simulink subsystem "PowerSystemRefAeronomie"  (R2024b)
settings: Solver=VariableStepAuto  StartTime=0.0  StopTime=10.0  RelTol=1e-3
undefined symbols (not defined in the file or in its folder): ess, mot, powerplant, propel, pxf_diagram_options, SimIn, tc
libraries: simulink x2, slpidlib x1, matrix_library x1
(part 1 of 3)
settings Model: Creator=drhill  LastModifiedBy=edison
settings SolverCC: AlgebraicLoopSolver=TrustRegion
settings OptimizationCC: ReuseModelBlockBuffer=off
settings DebuggingCC: UnconnectedInputMsg=warning  UnconnectedOutputMsg=warning  UnconnectedLineMsg=warning
settings ModelReferenceCC: EnableRefExpFcnMdlSchedulingChecks=on
settings RTWCC: GPUComputeCapability=3.5  DLArmComputeVersion=19.05

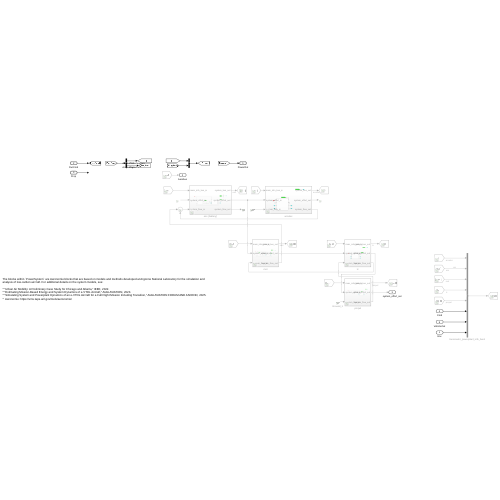
[thumbnail: Simulink's stored preview of the top-level diagram]
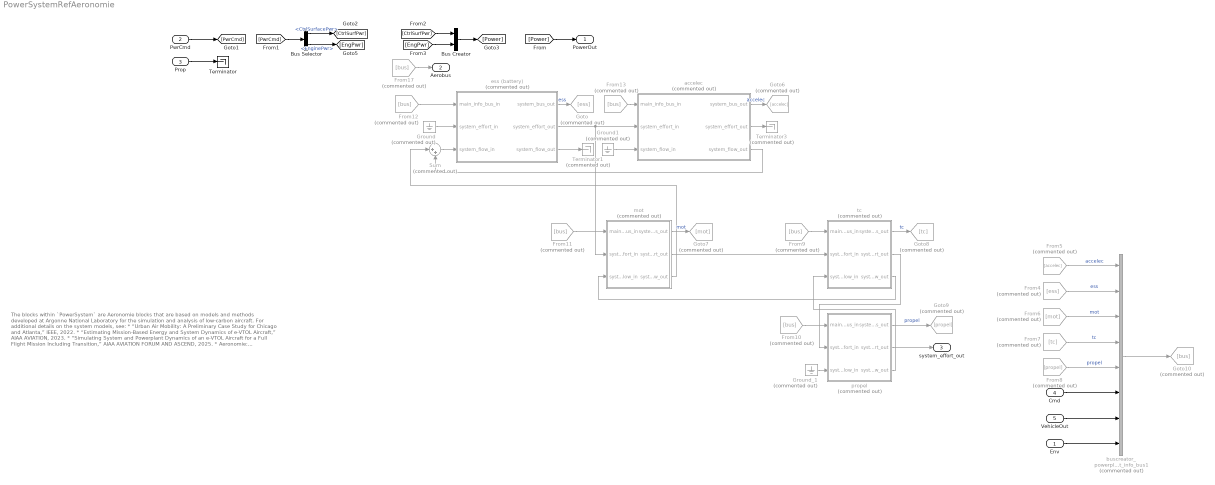
== system PowerSystemRefAeronomie ==
  note: The blocks within `PowerSystem` are Aeronomie blocks that are based on models and methods developed at Argonne National Laboratory for the simulation and analysis of low-carbon aircraft. For additional details on the system models, see:
      |
      | * “Urban Air Mobility: A Preliminary Case Study for Chicago and Atlanta,” IEEE, 2022.
      | * “Estimating Mission-Based Energy and System Dynamics of e-VTOL Aircraft,” AIAA AVIATION, 2023.
      | * “Simulating System and Powerplant Dynamics of an e-VTOL Aircraft for a Full Flight Mission Including Transition,” AIAA AVIATION FORUM AND ASCEND, 2025.
      | * Aeronomie: https://vms.taps.anl.gov/tools/aeronomie/
  Env : Inport
  PwrCmd : Inport  Port=2  OutDataTypeStr=Bus: BUS_POWER_SYSTEM_IN
  Prop : Inport  Port=3  OutDataTypeStr=Bus: BUS_PROP_ACTUATOR
  Cmd : Inport  Port=4
  VehicleOut : Inport  Port=5
  Bus Creator : BusCreator  Inputs=2  OutDataTypeStr=Bus: BUS_POWER_SYSTEM_OUT
  Bus Selector : BusSelector  OutputSignals=CtrlSurfacePwr,EnginePwr
  From{9..13,17} (6 alike) : From  Commented=on  GotoTag=bus
  From4 : From  Commented=on  GotoTag=ess
  From5 : From  Commented=on  GotoTag=accelec
  From6 : From  Commented=on  GotoTag=mot
  From7 : From  Commented=on  GotoTag=tc
  From8 : From  Commented=on  GotoTag=propel
  Goto : Goto  Commented=on  GotoTag=ess
  Goto10 : Goto  Commented=on  GotoTag=bus
  Goto6 : Goto  Commented=on  GotoTag=accelec
  Goto7 : Goto  Commented=on  GotoTag=mot
  Goto8 : Goto  Commented=on  GotoTag=tc
  Goto9 : Goto  Commented=on  GotoTag=propel
  Ground : Ground  Commented=on
  Ground1 : Ground  Commented=on
  Ground_1 : Ground  Commented=on
  Sum : Sum  Commented=on  Inputs=|++
  Terminator : Terminator
  Terminator1 : Terminator  Commented=on
  Terminator3 : Terminator  Commented=on
  accelec : Subsystem  Commented=on
  buscreator_powerplant_info_bus1 : BusCreator  Commented=on  Inputs=8
  ess (battery) : Subsystem  Commented=on
  mot : Subsystem  Commented=on
  propel : Subsystem  Commented=on
  tc : Subsystem  Commented=on
  PowerOut : Outport  OutDataTypeStr=Bus: BUS_POWER_SYSTEM_OUT  VectorParamsAs1DForOutWhenUnconnected=off
  Aerobus : Outport  Port=2
  system_effort_out : Outport  Port=3
  wires:
  mot/2(system_effort_out) -> tc/2(system_effort_in)
  Ground_1/1 -> propel/3(system_flow_in)
  tc/3(system_flow_out) -> mot/3(system_flow_in)
  tc/2(system_effort_out) -> propel/2(system_effort_in)
  propel/3(system_flow_out) -> tc/3(system_flow_in)
  Bus Creator/1 -> [Power]
  [Power] -> PowerOut/1
  PwrCmd/1 -> [PwrCmd]
  [PwrCmd] -> Bus Selector/1
  Bus Selector/1 -> [CtrlSurfPwr]  "<CtrlSurfacePwr>"
  [CtrlSurfPwr] -> Bus Creator/1
  [EngPwr] -> Bus Creator/2
  Ground/1 -> ess (battery)/2(system_effort_in)
  Prop/1 -> Terminator/1
  ess (battery)/3(system_flow_out) -> Terminator1/1
  Bus Selector/2 -> [EngPwr]  "<EnginePwr>"
  ess (battery)/2(system_effort_out) -> mot/2(system_effort_in), accelec/2(system_effort_in)
  Ground1/1 -> accelec/3(system_flow_in)
  Sum/1 -> ess (battery)/3(system_flow_in)
  accelec/3(system_flow_out) -> Sum/2
  accelec/2(system_effort_out) -> Terminator3/1
  accelec/1(system_bus_out) -> Goto6/1  "accelec"
  From5/1 -> buscreator_powerplant_info_bus1/1  "accelec"
  From4/1 -> buscreator_powerplant_info_bus1/2  "ess"
  From6/1 -> buscreator_powerplant_info_bus1/3  "mot"
  mot/1(system_bus_out) -> Goto7/1  "mot"
  tc/1(system_bus_out) -> Goto8/1  "tc"
  propel/1(system_bus_out) -> Goto9/1  "propel"
  From7/1 -> buscreator_powerplant_info_bus1/4  "tc"
  From8/1 -> buscreator_powerplant_info_bus1/5  "propel"
  From9/1 -> tc/1(main_info_bus_in)
  From10/1 -> propel/1(main_info_bus_in)
  From11/1 -> mot/1(main_info_bus_in)
  Cmd/1 -> buscreator_powerplant_info_bus1/6
  Env/1 -> buscreator_powerplant_info_bus1/8
  From12/1 -> ess (battery)/1(main_info_bus_in)
  From13/1 -> accelec/1(main_info_bus_in)
  ess (battery)/1(system_bus_out) -> Goto/1  "ess"
  propel/2(system_effort_out) -> system_effort_out/1
  From17/1 -> Aerobus/1
  VehicleOut/1 -> buscreator_powerplant_info_bus1/7
  buscreator_powerplant_info_bus1/1 -> Goto10/1
  mot/3(system_flow_out) -> Sum/1

== system PowerSystemRefAeronomie/accelec ==
  main_info_bus_in : Inport
  system_effort_in : Inport  Port=2
  system_flow_in : Inport  Port=3
  Ground_1 : Ground
  Terminator_1 : Terminator
  plant : Subsystem
      mask Display: disp('accelec_plant_const_pwrloss_volt_in_nokey.slx')
  system_bus_out : Outport
  system_effort_out : Outport  Port=2
  system_flow_out : Outport  Port=3
  wires:
  main_info_bus_in/1 -> plant/1(aInport--1)
  plant/1(outport-system_info_bus) -> [plant]
  plant/3(out-effort-6) -> system_effort_out/1
  plant/4(out-flow-7) -> system_flow_out/1
  system_effort_in/1 -> plant/3(in-effort-2)
  system_flow_in/1 -> plant/4(in-flow-3)
  [plant] -> system_bus_out/1  "plant"
  Ground_1/1 -> plant/2(aInport--2)
  plant/2(aOutport--2) -> Terminator_1/1

== system PowerSystemRefAeronomie/ess (battery) ==
  main_info_bus_in : Inport
  system_effort_in : Inport  Port=2
  system_flow_in : Inport  Port=3
  buscreator_system_bus_out1 : BusCreator  Inputs=2
  ctrl : Subsystem
      mask Display: disp('ess_ctrl_pngv_map_anl_PI_cstr.slx')
  memoryctrl : Memory
  plant : Subsystem
      mask Display: disp('ess_plant_pngv_map_anl_PI_cstr.slx')
  system_bus_out : Outport
  system_effort_out : Outport  Port=2
  system_flow_out : Outport  Port=3
  wires:
  ctrl/1(outport-system_info_bus) -> [ctrl]  "system_info_bus"
  ctrl/2(outport-ctrl_bus) -> memoryctrl/1  "ctrl_bus"
  main_info_bus_in/1 -> ctrl/1(inport-main_info_bus-1), plant/1(aInport--1)  "main_info_bus"
  plant/2(outport-plant_bus) -> ctrl/2(aInport--2)  "plant_bus"
  memoryctrl/1 -> plant/2(aInport--2)  "ctrl_bus"
  plant/1(outport-system_info_bus) -> [plant]  "system_info_bus"
  plant/3(out-effort-12) -> system_effort_out/1  "effort"
  plant/4(out-flow-13) -> system_flow_out/1  "flow"
  system_effort_in/1 -> plant/3(in-effort-1)  "effort"
  system_flow_in/1 -> plant/4(in-flow-2)  "flow"
  buscreator_system_bus_out1/1 -> system_bus_out/1  "system_info_bus"
  [ctrl] -> buscreator_system_bus_out1/1  "ctrl"
  [plant] -> buscreator_system_bus_out1/2  "plant"

== system PowerSystemRefAeronomie/mot ==
  main_info_bus_in : Inport
  system_effort_in : Inport  Port=2
  system_flow_in : Inport  Port=3
  buscreator_system_bus_out1 : BusCreator  Inputs=2
  ctrl : Subsystem
  memoryctrl : Memory
  plant : Subsystem
      mask Display: disp('mot_plant_map_Pelec_funTW_volt_in.slx')
  system_bus_out : Outport
  system_effort_out : Outport  Port=2
  system_flow_out : Outport  Port=3
  wires:
  ctrl/1(system_bus_out) -> [ctrl]  "system_info_bus"
  ctrl/2(local_info_bus_out) -> memoryctrl/1  "ctrl_bus"
  main_info_bus_in/1 -> ctrl/1(main_info_bus_in), plant/1(aInport--1)  "main_info_bus"
  plant/2(outport-plant_bus) -> ctrl/2(local_info_bus_in)  "plant_bus"
  memoryctrl/1 -> plant/2(inport-ctrl_bus-2)  "ctrl_bus"
  plant/1(outport-system_info_bus) -> [plant]  "system_info_bus"
  plant/3(out-effort-7) -> system_effort_out/1  "effort"
  plant/4(out-flow-8) -> system_flow_out/1  "flow"
  system_effort_in/1 -> plant/3(in-effort-2)  "effort"
  system_flow_in/1 -> plant/4(in-flow-3)  "flow"
  buscreator_system_bus_out1/1 -> system_bus_out/1  "system_info_bus"
  [ctrl] -> buscreator_system_bus_out1/1  "ctrl"
  [plant] -> buscreator_system_bus_out1/2  "plant"

== system PowerSystemRefAeronomie/propel ==
  main_info_bus_in : Inport
  system_effort_in : Inport  Port=2
  system_flow_in : Inport  Port=3
  Ground_1 : Ground
  Terminator_1 : Terminator
  plant : Subsystem
      mask Display: disp('propel_plant_uas.slx')
  system_bus_out : Outport
  system_effort_out : Outport  Port=2
  system_flow_out : Outport  Port=3
  wires:
  main_info_bus_in/1 -> plant/1(inport-main_info_bus-1)
  plant/1(outport-system_info_bus) -> [plant]
  plant/3(out-effort-5) -> system_effort_out/1
  plant/4(out-flow-6) -> system_flow_out/1
  system_effort_in/1 -> plant/3(in-effort-4)
  system_flow_in/1 -> plant/4(in-flow-5)
  [plant] -> system_bus_out/1  "plant"
  Ground_1/1 -> plant/2(aInport--2)
  plant/2(aOutport--2) -> Terminator_1/1

== system PowerSystemRefAeronomie/tc ==
  main_info_bus_in : Inport
  system_effort_in : Inport  Port=2
  system_flow_in : Inport  Port=3
  Ground_1 : Ground
  Terminator_1 : Terminator
  plant : Subsystem
      mask Display: disp('tc_plant_map_trqloss_funTW.slx')
  system_bus_out : Outport
  system_effort_out : Outport  Port=2
  system_flow_out : Outport  Port=3
  wires:
  main_info_bus_in/1 -> plant/1(aInport--1)
  plant/1(outport-system_info_bus) -> [plant]
  plant/3(out-effort-7) -> system_effort_out/1
  plant/4(out-flow-8) -> system_flow_out/1
  system_effort_in/1 -> plant/3(in-effort-1)
  system_flow_in/1 -> plant/4(in-flow-2)
  [plant] -> system_bus_out/1  "plant"
  Ground_1/1 -> plant/2(aInport--2)
  plant/2(aOutport--2) -> Terminator_1/1

== system PowerSystemRefAeronomie/accelec/plant ==
  aInport--1 : Inport
  aInport--2 : Inport  Port=2
  in-effort-2 : Inport  Port=3
  in-flow-3 : Inport  Port=4
  Ground_1 : Ground
  Ground_2 : Ground
  Terminator_1 : Terminator
  Terminator_2 : Terminator
  accelec_plant_const_pwrloss_volt_in_nokey : Subsystem
  parameter_out : Subsystem
  parameter_selection : Subsystem
  outport-system_info_bus : Outport
  aOutport--2 : Outport  Port=2
  out-effort-6 : Outport  Port=3
  out-flow-7 : Outport  Port=4
  wires:
  parameter_out/1(outport-system_info_bus) -> outport-system_info_bus/1
  accelec_plant_const_pwrloss_volt_in_nokey/1(accelec_plant_volt_in_simu) -> parameter_out/1(inport-accelec_plant_volt_in_simu)
  accelec_plant_const_pwrloss_volt_in_nokey/2(accelec_plant_pwr_simu) -> parameter_out/2(inport-accelec_plant_pwr_simu)
  accelec_plant_const_pwrloss_volt_in_nokey/3(accelec_plant_curr_in_simu) -> parameter_out/3(inport-accelec_plant_curr_in_simu)
  accelec_plant_const_pwrloss_volt_in_nokey/4(accelec_plant_volt_out_simu) -> parameter_out/4(inport-accelec_plant_volt_out_simu)
  accelec_plant_const_pwrloss_volt_in_nokey/5(accelec_plant_curr_out_simu) -> parameter_out/5(inport-accelec_plant_curr_out_simu)
  in-effort-2/1 -> accelec_plant_const_pwrloss_volt_in_nokey/2(accelec_volt_in)
  in-flow-3/1 -> accelec_plant_const_pwrloss_volt_in_nokey/3(accelec_curr_out)
  accelec_plant_const_pwrloss_volt_in_nokey/6(accelec_volt_out) -> out-effort-6/1
  accelec_plant_const_pwrloss_volt_in_nokey/7(accelec_curr_in) -> out-flow-7/1
  aInport--1/1 -> Terminator_1/1
  aInport--2/1 -> Terminator_2/1
  Ground_1/1 -> accelec_plant_const_pwrloss_volt_in_nokey/1(drv_key_on_dmd_simu)
  Ground_2/1 -> aOutport--2/1

== system PowerSystemRefAeronomie/ess (battery)/ctrl ==
  inport-main_info_bus-1 : Inport
  aInport--2 : Inport  Port=2
  Terminator_1 : Terminator
  ess_ctrl_pngv_map_anl_PI_cstr : Subsystem
  parameter_out : Subsystem
  parameter_selection : Subsystem
  outport-system_info_bus : Outport
  outport-ctrl_bus : Outport  Port=2
  wires:
  inport-main_info_bus-1/1 -> parameter_selection/1(inport-main_info_bus-1)
  parameter_out/1(outport-system_info_bus) -> outport-system_info_bus/1
  parameter_out/2(outport-ctrl_bus) -> outport-ctrl_bus/1
  ess_ctrl_pngv_map_anl_PI_cstr/1(ess_ctrl_pwr_max_pro_simu) -> parameter_out/1(inport-ess_ctrl_pwr_max_pro_simu)
  ess_ctrl_pngv_map_anl_PI_cstr/2(ess_ctrl_pwr_max_reg_simu) -> parameter_out/2(inport-ess_ctrl_pwr_max_reg_simu)
  ess_ctrl_pngv_map_anl_PI_cstr/3(ess_ctrl_curr_max_pro_simu) -> parameter_out/3(inport-ess_ctrl_curr_max_pro_simu)
  ess_ctrl_pngv_map_anl_PI_cstr/4(ess_ctrl_curr_max_reg_simu) -> parameter_out/4(inport-ess_ctrl_curr_max_reg_simu)
  parameter_selection/1(outport-ess_plant_volt_out_simu-1) -> ess_ctrl_pngv_map_anl_PI_cstr/1(ess_volt_out)
  parameter_selection/2(outport-ess_plant_curr_out_simu-2) -> ess_ctrl_pngv_map_anl_PI_cstr/2(ess_curr_out)
  parameter_selection/3(outport-ess_plant_soc_simu-3) -> ess_ctrl_pngv_map_anl_PI_cstr/3(ess_soc)
  aInport--2/1 -> Terminator_1/1

== system PowerSystemRefAeronomie/ess (battery)/plant ==
  aInport--1 : Inport
  aInport--2 : Inport  Port=2
  in-effort-1 : Inport  Port=3
  in-flow-2 : Inport  Port=4
  Terminator_1 : Terminator
  Terminator_2 : Terminator
  ess_plant_pngv_map_anl_PI_cstr : Subsystem
  parameter_out : Subsystem
  parameter_selection : Subsystem
  outport-system_info_bus : Outport
  outport-plant_bus : Outport  Port=2
  out-effort-12 : Outport  Port=3
  out-flow-13 : Outport  Port=4
  wires:
  parameter_out/1(outport-system_info_bus) -> outport-system_info_bus/1
  parameter_out/2(outport-plant_bus) -> outport-plant_bus/1
  ess_plant_pngv_map_anl_PI_cstr/1(ess_plant_soc_simu) -> parameter_out/1(inport-ess_plant_soc_simu)
  ess_plant_pngv_map_anl_PI_cstr/10(ess_plant_heat_out_simu) -> parameter_out/10(inport-ess_plant_heat_out_simu)
  ess_plant_pngv_map_anl_PI_cstr/11(ess_plant_impedance_simu) -> parameter_out/11(inport-ess_plant_impedance_simu)
  ess_plant_pngv_map_anl_PI_cstr/2(ess_plant_curr_out_simu) -> parameter_out/2(inport-ess_plant_curr_out_simu)
  ess_plant_pngv_map_anl_PI_cstr/3(ess_plant_volt_out_simu) -> parameter_out/3(inport-ess_plant_volt_out_simu)
  ess_plant_pngv_map_anl_PI_cstr/4(ess_plant_voc_simu) -> parameter_out/4(inport-ess_plant_voc_simu)
  ess_plant_pngv_map_anl_PI_cstr/5(ess_plant_rint_simu) -> parameter_out/5(inport-ess_plant_rint_simu)
  ess_plant_pngv_map_anl_PI_cstr/6(ess_plant_rpol1_simu) -> parameter_out/6(inport-ess_plant_rpol1_simu)
  ess_plant_pngv_map_anl_PI_cstr/7(ess_plant_rpol2_simu) -> parameter_out/7(inport-ess_plant_rpol2_simu)
  ess_plant_pngv_map_anl_PI_cstr/8(ess_plant_curr_pol1_simu) -> parameter_out/8(inport-ess_plant_curr_pol1_simu)
  ess_plant_pngv_map_anl_PI_cstr/9(ess_plant_curr_pol2_simu) -> parameter_out/9(inport-ess_plant_curr_pol2_simu)
  in-effort-1/1 -> ess_plant_pngv_map_anl_PI_cstr/1(ess_volt_in)
  in-flow-2/1 -> ess_plant_pngv_map_anl_PI_cstr/2(ess_curr_out)
  ess_plant_pngv_map_anl_PI_cstr/12(ess_volt_out) -> out-effort-12/1
  ess_plant_pngv_map_anl_PI_cstr/13(ess_curr_in) -> out-flow-13/1
  aInport--1/1 -> Terminator_1/1
  aInport--2/1 -> Terminator_2/1

== system PowerSystemRefAeronomie/mot/ctrl ==
  main_info_bus_in : Inport
  local_info_bus_in : Inport  Port=2
  buscreator_system_bus_out1 : BusCreator  Inputs=3
  cmd : Subsystem
      mask Display: disp('mot_ctrl_cmd_map_Pelec_funTW_volt_in.slx')
  cstr : Subsystem
      mask Display: disp('mot_ctrl_cstr_map_Pelec_funTW_volt_in.slx')
  dmd : Subsystem
      mask Display: disp('mot_ctrl_dmd_uas.slx')
  system_bus_out : Outport
  local_info_bus_out : Outport  Port=2
  wires:
  dmd/1(outport-system_info_bus) -> [dmd]
  dmd/2(outport-dmd_bus) -> cmd/4(aInport--4), cstr/3(aInport--3)
  [local_info_bus] -> dmd/2(aInport--2)
  [main_info_bus] -> dmd/1(inport-main_info_bus-1)
  cstr/1(outport-system_info_bus) -> [cstr]
  cstr/2(outport-cstr_bus) -> cmd/3(aInport--3)
  [local_info_bus] -> cstr/2(aInport--2)
  [main_info_bus] -> cstr/1(inport-main_info_bus-1)
  cmd/1(outport-system_info_bus) -> local_info_bus_out/1, [cmd]
  [local_info_bus] -> cmd/2(aInport--2)
  [main_info_bus] -> cmd/1(inport-main_info_bus-1)
  main_info_bus_in/1 -> [main_info_bus]
  local_info_bus_in/1 -> [local_info_bus]
  buscreator_system_bus_out1/1 -> system_bus_out/1
  [cmd] -> buscreator_system_bus_out1/1  "cmd"
  [cstr] -> buscreator_system_bus_out1/2  "cstr"
  [dmd] -> buscreator_system_bus_out1/3  "dmd"

== system PowerSystemRefAeronomie/mot/plant ==
  aInport--1 : Inport
  inport-ctrl_bus-2 : Inport  Port=2
  in-effort-2 : Inport  Port=3
  in-flow-3 : Inport  Port=4
  Ground_1 : Ground
  Terminator_1 : Terminator
  mot_plant_map_Pelec_funTW_volt_in : Subsystem
  parameter_out : Subsystem
  parameter_selection : Subsystem
  outport-system_info_bus : Outport
  outport-plant_bus : Outport  Port=2
  out-effort-7 : Outport  Port=3
  out-flow-8 : Outport  Port=4
  wires:
  inport-ctrl_bus-2/1 -> parameter_selection/2(inport-ctrl_bus-2)
  parameter_out/1(outport-system_info_bus) -> outport-system_info_bus/1
  parameter_out/2(outport-plant_bus) -> outport-plant_bus/1
  mot_plant_map_Pelec_funTW_volt_in/1(mot_plant_spd_out_simu) -> parameter_out/1(inport-mot_plant_spd_out_simu)
  mot_plant_map_Pelec_funTW_volt_in/2(mot_plant_curr_in_simu) -> parameter_out/2(inport-mot_plant_curr_in_simu)
  mot_plant_map_Pelec_funTW_volt_in/3(mot_plant_volt_in_simu) -> parameter_out/3(inport-mot_plant_volt_in_simu)
  mot_plant_map_Pelec_funTW_volt_in/4(mot_plant_cmd_simu) -> parameter_out/4(inport-mot_plant_cmd_simu)
  mot_plant_map_Pelec_funTW_volt_in/5(mot_plant_trq_out_simu) -> parameter_out/5(inport-mot_plant_trq_out_simu)
  mot_plant_map_Pelec_funTW_volt_in/6(mot_plant_temp_coeff_simu) -> parameter_out/6(inport-mot_plant_temp_coeff_simu)
  parameter_selection/1(outport-mot_ctrl_cmd_simu-1) -> mot_plant_map_Pelec_funTW_volt_in/1(mot_ctrl_cmd_simu)
  in-effort-2/1 -> mot_plant_map_Pelec_funTW_volt_in/2(voltage)
  in-flow-3/1 -> mot_plant_map_Pelec_funTW_volt_in/3(spd)
  mot_plant_map_Pelec_funTW_volt_in/7(mot_trq_out mot_inertia_out) -> out-effort-7/1
  mot_plant_map_Pelec_funTW_volt_in/8(mot_current_out) -> out-flow-8/1
  aInport--1/1 -> Terminator_1/1
  Ground_1/1 -> parameter_selection/1(Inport_1)

== system PowerSystemRefAeronomie/propel/plant ==
  inport-main_info_bus-1 : Inport
  aInport--2 : Inport  Port=2
  in-effort-4 : Inport  Port=3
  in-flow-5 : Inport  Port=4
  Ground_1 : Ground
  Terminator_1 : Terminator
  parameter_out : Subsystem
  parameter_selection : Subsystem
  propel_plant_uas : Subsystem
  outport-system_info_bus : Outport
  aOutport--2 : Outport  Port=2
  out-effort-5 : Outport  Port=3
  out-flow-6 : Outport  Port=4
  wires:
  propel_plant_uas/7(propel_plant_effort_dn) -> parameter_out/6(propel_plant_effort_dn1)
  parameter_selection/4(tc_plant_trq_out_simu) -> propel_plant_uas/4(tc_plant_trq_out_simu)
  parameter_selection/5(AdvanceRatio) -> propel_plant_uas/6(AdvanceRatio)
  inport-main_info_bus-1/1 -> parameter_selection/1(inport-main_info_bus-1)
  parameter_out/1(outport-system_info_bus) -> outport-system_info_bus/1
  propel_plant_uas/1(propel_plant_speed_simu) -> parameter_out/1(inport-propel_plant_speed_simu)
  propel_plant_uas/2(propel_plant_pwr_in_simu) -> parameter_out/2(inport-propel_plant_pwr_in_simu)
  propel_plant_uas/3(propel_plant_pwr_out_simu) -> parameter_out/3(inport-propel_plant_pwr_out_simu)
  propel_plant_uas/4(propel_plant_thrust_simu) -> parameter_out/4(inport-propel_plant_thrust_simu)
  parameter_selection/1(outport-env_plant_density_simu-1) -> propel_plant_uas/1(env_plant_density_simu)
  parameter_selection/2(outport-tc_plant_inertia_out_simu-2) -> propel_plant_uas/2(tc_plant_inertia_out_simu)
  parameter_selection/3(outport-eqnmotion_plant_linvel_simu-3) -> propel_plant_uas/3(eqnmotion_plant_linvel_simu)
  in-flow-5/1 -> propel_plant_uas/5(flow-in)
  propel_plant_uas/5(propel_plant_effort) -> out-effort-5/1, parameter_out/5(propel_plant_effort)
  propel_plant_uas/6(propel_plant_speed_out_simu) -> out-flow-6/1
  aInport--2/1 -> Terminator_1/1
  Ground_1/1 -> aOutport--2/1

== system PowerSystemRefAeronomie/tc/plant ==
  aInport--1 : Inport
  aInport--2 : Inport  Port=2
  in-effort-1 : Inport  Port=3
  in-flow-2 : Inport  Port=4
  Ground_1 : Ground
  Terminator_1 : Terminator
  Terminator_2 : Terminator
  parameter_out : Subsystem
  parameter_selection : Subsystem
  tc_plant_map_trqloss_funTW : Subsystem
  outport-system_info_bus : Outport
  aOutport--2 : Outport  Port=2
  out-effort-7 : Outport  Port=3
  out-flow-8 : Outport  Port=4
  wires:
  parameter_out/1(outport-system_info_bus) -> outport-system_info_bus/1
  tc_plant_map_trqloss_funTW/1(tc_plant_trq_in_simu) -> parameter_out/1(inport-tc_plant_trq_in_simu)
  tc_plant_map_trqloss_funTW/2(tc_plant_trq_out_simu) -> parameter_out/2(inport-tc_plant_trq_out_simu)
  tc_plant_map_trqloss_funTW/3(tc_plant_spd_in_simu) -> parameter_out/3(inport-tc_plant_spd_in_simu)
  tc_plant_map_trqloss_funTW/4(tc_plant_spd_out_simu) -> parameter_out/4(inport-tc_plant_spd_out_simu)
  tc_plant_map_trqloss_funTW/5(tc_plant_inertia_in_simu) -> parameter_out/5(inport-tc_plant_inertia_in_simu)
  tc_plant_map_trqloss_funTW/6(tc_plant_inertia_out_simu) -> parameter_out/6(inport-tc_plant_inertia_out_simu)
  in-effort-1/1 -> tc_plant_map_trqloss_funTW/1(tc_trq_in tc_inertia_in)
  in-flow-2/1 -> tc_plant_map_trqloss_funTW/2(tc_spd_out)
  tc_plant_map_trqloss_funTW/7(tc_trq_out) -> out-effort-7/1
  tc_plant_map_trqloss_funTW/8(tc_spd_in) -> out-flow-8/1
  aInport--2/1 -> Terminator_2/1
  Ground_1/1 -> aOutport--2/1
  aInport--1/1 -> Terminator_1/1

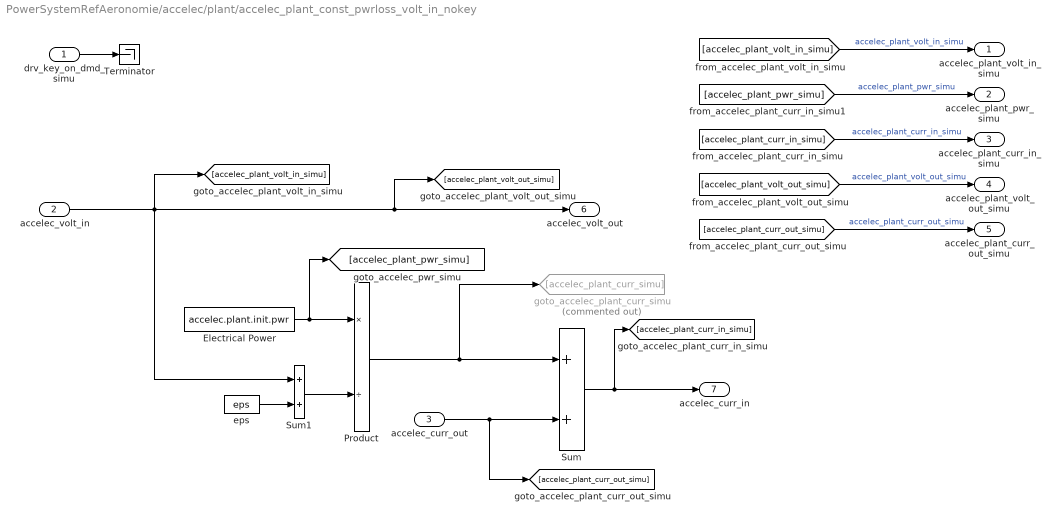
== system PowerSystemRefAeronomie/accelec/plant/accelec_plant_const_pwrloss_volt_in_nokey ==
  drv_key_on_dmd_simu : Inport
  accelec_volt_in : Inport  Port=2
  accelec_curr_out : Inport  Port=3
  Electrical Power : Constant  Value=accelec.plant.init.pwr
  Product : Product  Inputs=*/  InputSameDT=on  SaturateOnIntegerOverflow=on  OutDataTypeStr=Inherit: Same as first input
  Sum : Sum  InputSameDT=on  SaturateOnIntegerOverflow=on  OutDataTypeStr=Inherit: Same as first input
  Sum1 : Sum  InputSameDT=on  SaturateOnIntegerOverflow=on  OutDataTypeStr=Inherit: Same as first input
  Terminator : Terminator
  eps : Constant  Value=eps
  goto_accelec_plant_curr_simu : Goto  Commented=on  GotoTag=accelec_plant_curr_simu
  accelec_plant_volt_in_simu : Outport  VectorParamsAs1DForOutWhenUnconnected=off
  accelec_plant_pwr_simu : Outport  Port=2  VectorParamsAs1DForOutWhenUnconnected=off
  accelec_plant_curr_in_simu : Outport  Port=3  VectorParamsAs1DForOutWhenUnconnected=off
  accelec_plant_volt_out_simu : Outport  Port=4  VectorParamsAs1DForOutWhenUnconnected=off
  accelec_plant_curr_out_simu : Outport  Port=5  VectorParamsAs1DForOutWhenUnconnected=off
  accelec_volt_out : Outport  Port=6  VectorParamsAs1DForOutWhenUnconnected=off
  accelec_curr_in : Outport  Port=7  VectorParamsAs1DForOutWhenUnconnected=off
  wires:
  drv_key_on_dmd_simu/1 -> Terminator/1
  Electrical Power/1 -> Product/1, [accelec_plant_pwr_simu]
  [accelec_plant_volt_out_simu] -> accelec_plant_volt_out_simu/1  "accelec_plant_volt_out_simu"
  [accelec_plant_curr_out_simu] -> accelec_plant_curr_out_simu/1  "accelec_plant_curr_out_simu"
  [accelec_plant_curr_in_simu] -> accelec_plant_curr_in_simu/1  "accelec_plant_curr_in_simu"
  Sum1/1 -> Product/2
  Sum/1 -> accelec_curr_in/1, [accelec_plant_curr_in_simu]
  accelec_curr_out/1 -> Sum/2, [accelec_plant_curr_out_simu]
  Product/1 -> Sum/1, goto_accelec_plant_curr_simu/1
  eps/1 -> Sum1/2
  [accelec_plant_volt_in_simu] -> accelec_plant_volt_in_simu/1  "accelec_plant_volt_in_simu"
  accelec_volt_in/1 -> accelec_volt_out/1, [accelec_plant_volt_out_simu], [accelec_plant_volt_in_simu], Sum1/1
  [accelec_plant_pwr_simu] -> accelec_plant_pwr_simu/1  "accelec_plant_pwr_simu"

== system PowerSystemRefAeronomie/accelec/plant/parameter_out ==
  inport-accelec_plant_volt_in_simu : Inport
  inport-accelec_plant_pwr_simu : Inport  Port=2
  inport-accelec_plant_curr_in_simu : Inport  Port=3
  inport-accelec_plant_volt_out_simu : Inport  Port=4
  inport-accelec_plant_curr_out_simu : Inport  Port=5
  Ground_1 : Ground
  Toworkspace-accelec_plant_curr_in_simu : ToWorkspace  VariableName=accelec_plant_curr_in_simu  SampleTime=pxf_diagram_options.workspace_sample_time
      settings: Decimation=pxf_diagram_options.decimation
  Toworkspace-accelec_plant_curr_out_simu : ToWorkspace  VariableName=accelec_plant_curr_out_simu  SampleTime=pxf_diagram_options.workspace_sample_time
      settings: Decimation=pxf_diagram_options.decimation
  Toworkspace-accelec_plant_pwr_simu : ToWorkspace  VariableName=accelec_plant_pwr_simu  SampleTime=pxf_diagram_options.workspace_sample_time
      settings: Decimation=pxf_diagram_options.decimation
  Toworkspace-accelec_plant_volt_in_simu : ToWorkspace  VariableName=accelec_plant_volt_in_simu  SampleTime=pxf_diagram_options.workspace_sample_time
      settings: Decimation=pxf_diagram_options.decimation
  Toworkspace-accelec_plant_volt_out_simu : ToWorkspace  VariableName=accelec_plant_volt_out_simu  SampleTime=pxf_diagram_options.workspace_sample_time
      settings: Decimation=pxf_diagram_options.decimation
  outport-system_info_bus : Outport
  wires:
  inport-accelec_plant_volt_in_simu/1 -> Toworkspace-accelec_plant_volt_in_simu/1
  inport-accelec_plant_pwr_simu/1 -> Toworkspace-accelec_plant_pwr_simu/1
  inport-accelec_plant_curr_in_simu/1 -> Toworkspace-accelec_plant_curr_in_simu/1
  inport-accelec_plant_volt_out_simu/1 -> Toworkspace-accelec_plant_volt_out_simu/1
  inport-accelec_plant_curr_out_simu/1 -> Toworkspace-accelec_plant_curr_out_simu/1
  Ground_1/1 -> outport-system_info_bus/1

== system PowerSystemRefAeronomie/accelec/plant/parameter_selection ==

== system PowerSystemRefAeronomie/ess (battery)/ctrl/ess_ctrl_pngv_map_anl_PI_cstr ==
  ess_volt_out : Inport
  ess_curr_out : Inport  Port=2
  ess_soc : Inport  Port=3
  Demux : Demux  Outputs=3
  Demux1 : Demux  Outputs=3
  PI controller for maximal charge power and current1 : Subsystem
  PI controller for maximal discharge power and current1 : Subsystem
  mux1 : Mux  Inputs=3
  ess_ctrl_pwr_max_pro_simu : Outport
  ess_ctrl_pwr_max_reg_simu : Outport  Port=2
  ess_ctrl_curr_max_pro_simu : Outport  Port=3
  ess_ctrl_curr_max_reg_simu : Outport  Port=4
  wires:
  ess_soc/1 -> mux1/3  "ess_plant_soc_simu"
  ess_curr_out/1 -> mux1/2  "ess_plant_curr_out_simu"
  Demux1/3 -> PI controller for maximal charge power and current1/3(SOC)
  Demux1/2 -> PI controller for maximal charge power and current1/2(ess curr)
  Demux1/1 -> PI controller for maximal charge power and current1/1(ess voltage)
  Demux/3 -> PI controller for maximal discharge power and current1/3(SOC)
  Demux/2 -> PI controller for maximal discharge power and current1/2(ess curr)
  Demux/1 -> PI controller for maximal discharge power and current1/1(ess voltage)
  PI controller for maximal charge power and current1/1(Pwr_max_reg) -> [ess_ctrl_pwr_max_reg_simu]
  PI controller for maximal discharge power and current1/2(Pwr_max_prop) -> [ess_ctrl_pwr_max_pro_simu]
  mux1/1 -> Demux1/1, Demux/1
  ess_volt_out/1 -> mux1/1  "ess_plant_volt_out_simu"
  PI controller for maximal charge power and current1/2(Curr_max_reg) -> [ess_ctrl_curr_max_reg_simu]
  PI controller for maximal discharge power and current1/1(Curr_max_prop) -> [ess_ctrl_curr_max_pro_simu]
  [ess_ctrl_curr_max_reg_simu] -> ess_ctrl_curr_max_reg_simu/1  "ess_ctrl_curr_max_reg_simu"
  [ess_ctrl_curr_max_pro_simu] -> ess_ctrl_curr_max_pro_simu/1  "ess_ctrl_curr_max_pro_simu"
  [ess_ctrl_pwr_max_pro_simu] -> ess_ctrl_pwr_max_pro_simu/1  "ess_ctrl_pwr_max_pro_simu"
  [ess_ctrl_pwr_max_reg_simu] -> ess_ctrl_pwr_max_reg_simu/1  "ess_ctrl_pwr_max_reg_simu"

== system PowerSystemRefAeronomie/ess (battery)/ctrl/parameter_out ==
  inport-ess_ctrl_pwr_max_pro_simu : Inport
  inport-ess_ctrl_pwr_max_reg_simu : Inport  Port=2
  inport-ess_ctrl_curr_max_pro_simu : Inport  Port=3
  inport-ess_ctrl_curr_max_reg_simu : Inport  Port=4
  Ground_1 : Ground
  Toworkspace-ess_ctrl_curr_max_pro_simu : ToWorkspace  VariableName=ess_ctrl_curr_max_pro_simu  SampleTime=pxf_diagram_options.workspace_sample_time
      settings: Decimation=pxf_diagram_options.decimation
  Toworkspace-ess_ctrl_curr_max_reg_simu : ToWorkspace  VariableName=ess_ctrl_curr_max_reg_simu  SampleTime=pxf_diagram_options.workspace_sample_time
      settings: Decimation=pxf_diagram_options.decimation
  Toworkspace-ess_ctrl_pwr_max_pro_simu : ToWorkspace  VariableName=ess_ctrl_pwr_max_pro_simu  SampleTime=pxf_diagram_options.workspace_sample_time
      settings: Decimation=pxf_diagram_options.decimation
  Toworkspace-ess_ctrl_pwr_max_reg_simu : ToWorkspace  VariableName=ess_ctrl_pwr_max_reg_simu  SampleTime=pxf_diagram_options.workspace_sample_time
      settings: Decimation=pxf_diagram_options.decimation
  create_system_info_bus : BusCreator  Inputs=1
  outport-system_info_bus : Outport
  outport-ctrl_bus : Outport  Port=2
  wires:
  create_system_info_bus/1 -> outport-system_info_bus/1
  inport-ess_ctrl_pwr_max_pro_simu/1 -> create_system_info_bus/1, Toworkspace-ess_ctrl_pwr_max_pro_simu/1  "ess_ctrl_pwr_max_pro_simu"
  inport-ess_ctrl_pwr_max_reg_simu/1 -> Toworkspace-ess_ctrl_pwr_max_reg_simu/1
  inport-ess_ctrl_curr_max_pro_simu/1 -> Toworkspace-ess_ctrl_curr_max_pro_simu/1
  inport-ess_ctrl_curr_max_reg_simu/1 -> Toworkspace-ess_ctrl_curr_max_reg_simu/1
  Ground_1/1 -> outport-ctrl_bus/1

== system PowerSystemRefAeronomie/ess (battery)/ctrl/parameter_selection ==
  inport-main_info_bus-1 : Inport
  select_main_info_bus : BusSelector  OutputSignals=ess.plant.ess_plant_volt_out_simu,ess.plant.ess_plant_curr_out_simu,ess.plant.ess_plant_soc_simu
  outport-ess_plant_volt_out_simu-1 : Outport
  outport-ess_plant_curr_out_simu-2 : Outport  Port=2
  outport-ess_plant_soc_simu-3 : Outport  Port=3
  wires:
  inport-main_info_bus-1/1 -> select_main_info_bus/1
  select_main_info_bus/1 -> outport-ess_plant_volt_out_simu-1/1  "<ess_plant_volt_out_simu>"
  select_main_info_bus/2 -> outport-ess_plant_curr_out_simu-2/1  "<ess_plant_curr_out_simu>"
  select_main_info_bus/3 -> outport-ess_plant_soc_simu-3/1  "<ess_plant_soc_simu>"

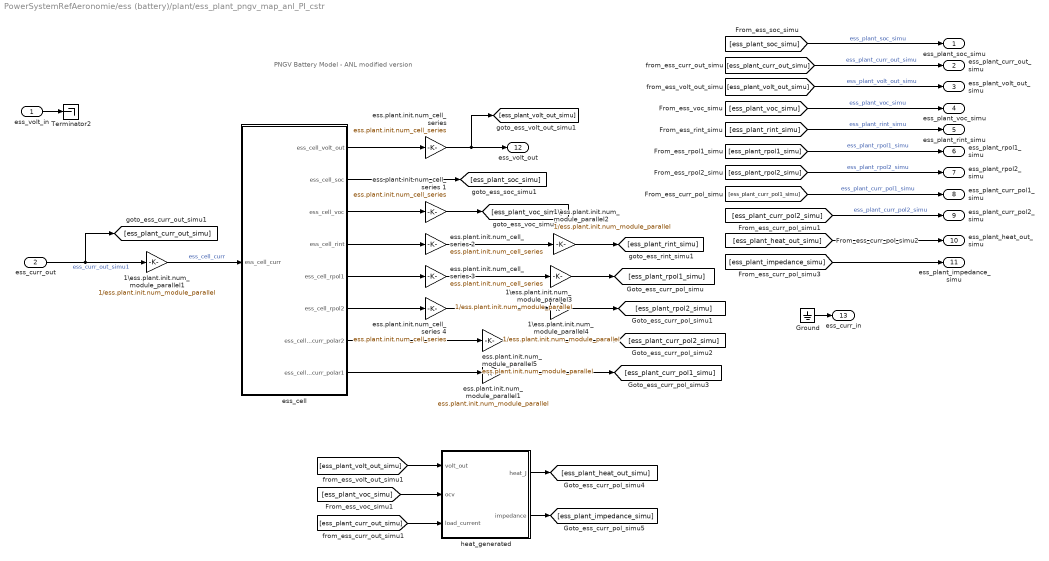
== system PowerSystemRefAeronomie/ess (battery)/plant/ess_plant_pngv_map_anl_PI_cstr ==
  note: PNGV Battery Model - ANL modified version
  ess_volt_in : Inport
  ess_curr_out : Inport  Port=2
  1\ess.plant.init.num_module_parallel{1..4} (4 alike) : Gain  Gain=1/ess.plant.init.num_module_parallel
  Ground : Ground
  Terminator2 : Terminator
  ess.plant.init.num_cell_series {,1..4} (5 alike) : Gain  Gain=ess.plant.init.num_cell_series
  ess.plant.init.num_module_parallel1 : Gain  Gain=ess.plant.init.num_module_parallel
  ess.plant.init.num_module_parallel5 : Gain  Gain=ess.plant.init.num_module_parallel
  ess_cell : Subsystem
  heat_generated : Subsystem
  ess_plant_soc_simu : Outport
  ess_plant_curr_out_simu : Outport  Port=2
  ess_plant_volt_out_simu : Outport  Port=3
  ess_plant_voc_simu : Outport  Port=4
  ess_plant_rint_simu : Outport  Port=5
  ess_plant_rpol1_simu : Outport  Port=6
  ess_plant_rpol2_simu : Outport  Port=7
  ess_plant_curr_pol1_simu : Outport  Port=8
  ess_plant_curr_pol2_simu : Outport  Port=9
  ess_plant_heat_out_simu : Outport  Port=10
  ess_plant_impedance_simu : Outport  Port=11
  ess_volt_out : Outport  Port=12
  ess_curr_in : Outport  Port=13
  wires:
  [ess_plant_impedance_simu] -> ess_plant_impedance_simu/1
  heat_generated/2(impedance) -> [ess_plant_impedance_simu]
  [ess_plant_heat_out_simu] -> ess_plant_heat_out_simu/1
  heat_generated/1(heat_J) -> [ess_plant_heat_out_simu]
  [ess_plant_curr_out_simu] -> heat_generated/3(load_current)
  [ess_plant_voc_simu] -> heat_generated/2(ocv)
  [ess_plant_volt_out_simu] -> heat_generated/1(volt_out)
  ess.plant.init.num_module_parallel1/1 -> [ess_plant_curr_pol1_simu]
  ess.plant.init.num_module_parallel5/1 -> [ess_plant_curr_pol2_simu]
  ess_cell/7(ess_cell_curr_polar2) -> ess.plant.init.num_module_parallel5/1
  ess_cell/8(ess_cell_curr_polar1) -> ess.plant.init.num_module_parallel1/1
  1\ess.plant.init.num_module_parallel4/1 -> [ess_plant_rpol2_simu]
  ess.plant.init.num_cell_series 4/1 -> 1\ess.plant.init.num_module_parallel4/1
  1\ess.plant.init.num_module_parallel3/1 -> [ess_plant_rpol1_simu]
  ess.plant.init.num_cell_series 3/1 -> 1\ess.plant.init.num_module_parallel3/1
  ess_cell/6(ess_cell_rpol2) -> ess.plant.init.num_cell_series 4/1
  ess_cell/5(ess_cell_rpol1) -> ess.plant.init.num_cell_series 3/1
  ess_cell/2(ess_cell_soc) -> [ess_plant_soc_simu]
  ess_cell/4(ess_cell_rint) -> ess.plant.init.num_cell_series 2/1
  ess_cell/3(ess_cell_voc) -> ess.plant.init.num_cell_series 1/1
  ess_curr_out/1 -> [ess_plant_curr_out_simu], 1\ess.plant.init.num_module_parallel1/1  "ess_curr_out_simu1"
  1\ess.plant.init.num_module_parallel2/1 -> [ess_plant_rint_simu]
  ess.plant.init.num_cell_series 1/1 -> [ess_plant_voc_simu]
  ess.plant.init.num_cell_series 2/1 -> 1\ess.plant.init.num_module_parallel2/1
  "ess.plant.init.num_cell_series "/1 -> ess_volt_out/1, [ess_plant_volt_out_simu]
  1\ess.plant.init.num_module_parallel1/1 -> ess_cell/1(ess_cell_curr)  "ess_cell_curr"
  ess_cell/1(ess_cell_volt_out) -> "ess.plant.init.num_cell_series "/1
  [ess_plant_curr_pol2_simu] -> ess_plant_curr_pol2_simu/1  "ess_plant_curr_pol2_simu"
  [ess_plant_curr_pol1_simu] -> ess_plant_curr_pol1_simu/1  "ess_plant_curr_pol1_simu"
  [ess_plant_rpol2_simu] -> ess_plant_rpol2_simu/1  "ess_plant_rpol2_simu"
  [ess_plant_rpol1_simu] -> ess_plant_rpol1_simu/1  "ess_plant_rpol1_simu"
  [ess_plant_rint_simu] -> ess_plant_rint_simu/1  "ess_plant_rint_simu"
  [ess_plant_voc_simu] -> ess_plant_voc_simu/1  "ess_plant_voc_simu"
  [ess_plant_volt_out_simu] -> ess_plant_volt_out_simu/1  "ess_plant_volt_out_simu"
  [ess_plant_curr_out_simu] -> ess_plant_curr_out_simu/1  "ess_plant_curr_out_simu"
  [ess_plant_soc_simu] -> ess_plant_soc_simu/1  "ess_plant_soc_simu"
  ess_volt_in/1 -> Terminator2/1
  Ground/1 -> ess_curr_in/1

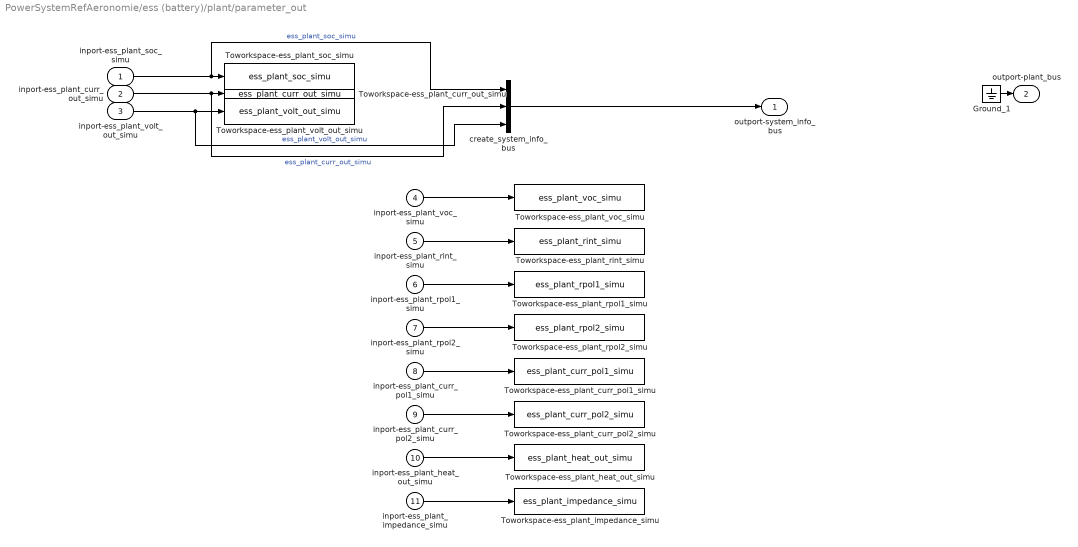
== system PowerSystemRefAeronomie/ess (battery)/plant/parameter_out ==
  inport-ess_plant_soc_simu : Inport
  inport-ess_plant_curr_out_simu : Inport  Port=2
  inport-ess_plant_volt_out_simu : Inport  Port=3
  inport-ess_plant_voc_simu : Inport  Port=4
  inport-ess_plant_rint_simu : Inport  Port=5
  inport-ess_plant_rpol1_simu : Inport  Port=6
  inport-ess_plant_rpol2_simu : Inport  Port=7
  inport-ess_plant_curr_pol1_simu : Inport  Port=8
  inport-ess_plant_curr_pol2_simu : Inport  Port=9
  inport-ess_plant_heat_out_simu : Inport  Port=10
  inport-ess_plant_impedance_simu : Inport  Port=11
  Ground_1 : Ground
  Toworkspace-ess_plant_curr_out_simu : ToWorkspace  VariableName=ess_plant_curr_out_simu  SampleTime=pxf_diagram_options.workspace_sample_time
      settings: Decimation=pxf_diagram_options.decimation
  Toworkspace-ess_plant_curr_pol1_simu : ToWorkspace  VariableName=ess_plant_curr_pol1_simu  SampleTime=pxf_diagram_options.workspace_sample_time
      settings: Decimation=pxf_diagram_options.decimation
  Toworkspace-ess_plant_curr_pol2_simu : ToWorkspace  VariableName=ess_plant_curr_pol2_simu  SampleTime=pxf_diagram_options.workspace_sample_time
      settings: Decimation=pxf_diagram_options.decimation
  Toworkspace-ess_plant_heat_out_simu : ToWorkspace  VariableName=ess_plant_heat_out_simu  SampleTime=pxf_diagram_options.workspace_sample_time
      settings: Decimation=pxf_diagram_options.decimation
  Toworkspace-ess_plant_impedance_simu : ToWorkspace  VariableName=ess_plant_impedance_simu  SampleTime=pxf_diagram_options.workspace_sample_time
      settings: Decimation=pxf_diagram_options.decimation
  Toworkspace-ess_plant_rint_simu : ToWorkspace  VariableName=ess_plant_rint_simu  SampleTime=pxf_diagram_options.workspace_sample_time
      settings: Decimation=pxf_diagram_options.decimation
  Toworkspace-ess_plant_rpol1_simu : ToWorkspace  VariableName=ess_plant_rpol1_simu  SampleTime=pxf_diagram_options.workspace_sample_time
      settings: Decimation=pxf_diagram_options.decimation
  Toworkspace-ess_plant_rpol2_simu : ToWorkspace  VariableName=ess_plant_rpol2_simu  SampleTime=pxf_diagram_options.workspace_sample_time
      settings: Decimation=pxf_diagram_options.decimation
  Toworkspace-ess_plant_soc_simu : ToWorkspace  VariableName=ess_plant_soc_simu  SampleTime=pxf_diagram_options.workspace_sample_time
      settings: Decimation=pxf_diagram_options.decimation
  Toworkspace-ess_plant_voc_simu : ToWorkspace  VariableName=ess_plant_voc_simu  SampleTime=pxf_diagram_options.workspace_sample_time
      settings: Decimation=pxf_diagram_options.decimation
  Toworkspace-ess_plant_volt_out_simu : ToWorkspace  VariableName=ess_plant_volt_out_simu  SampleTime=pxf_diagram_options.workspace_sample_time
      settings: Decimation=pxf_diagram_options.decimation
  create_system_info_bus : BusCreator  Inputs=3
  outport-system_info_bus : Outport
  outport-plant_bus : Outport  Port=2
  wires:
  create_system_info_bus/1 -> outport-system_info_bus/1
  inport-ess_plant_soc_simu/1 -> create_system_info_bus/1, Toworkspace-ess_plant_soc_simu/1  "ess_plant_soc_simu"
  inport-ess_plant_heat_out_simu/1 -> Toworkspace-ess_plant_heat_out_simu/1
  inport-ess_plant_impedance_simu/1 -> Toworkspace-ess_plant_impedance_simu/1
  inport-ess_plant_curr_out_simu/1 -> create_system_info_bus/2, Toworkspace-ess_plant_curr_out_simu/1  "ess_plant_curr_out_simu"
  inport-ess_plant_volt_out_simu/1 -> create_system_info_bus/3, Toworkspace-ess_plant_volt_out_simu/1  "ess_plant_volt_out_simu"
  inport-ess_plant_voc_simu/1 -> Toworkspace-ess_plant_voc_simu/1
  inport-ess_plant_rint_simu/1 -> Toworkspace-ess_plant_rint_simu/1
  inport-ess_plant_rpol1_simu/1 -> Toworkspace-ess_plant_rpol1_simu/1
  inport-ess_plant_rpol2_simu/1 -> Toworkspace-ess_plant_rpol2_simu/1
  inport-ess_plant_curr_pol1_simu/1 -> Toworkspace-ess_plant_curr_pol1_simu/1
  inport-ess_plant_curr_pol2_simu/1 -> Toworkspace-ess_plant_curr_pol2_simu/1
  Ground_1/1 -> outport-plant_bus/1

== system PowerSystemRefAeronomie/ess (battery)/plant/parameter_selection ==

== system PowerSystemRefAeronomie/mot/ctrl/cmd ==
  inport-main_info_bus-1 : Inport
  aInport--2 : Inport  Port=2
  aInport--3 : Inport  Port=3
  aInport--4 : Inport  Port=4
  Terminator_1 : Terminator
  Terminator_2 : Terminator
  Terminator_3 : Terminator
  mot_ctrl_cmd_map_Pelec_funTW_volt_in : Subsystem
  parameter_out : Subsystem
  parameter_selection : Subsystem
  outport-system_info_bus : Outport
  wires:
  inport-main_info_bus-1/1 -> parameter_selection/1(inport-main_info_bus-1)
  parameter_out/1(outport-system_info_bus) -> outport-system_info_bus/1
  mot_ctrl_cmd_map_Pelec_funTW_volt_in/1(mot_ctrl_cmd_simu) -> parameter_out/1(inport-mot_ctrl_cmd_simu)
  parameter_selection/1(outport-mot_plant_spd_out_simu-1) -> mot_ctrl_cmd_map_Pelec_funTW_volt_in/1(mot_plant_spd_out_simu)
  parameter_selection/2(outport-mot_ctrl_trs_trq_simu-2) -> mot_ctrl_cmd_map_Pelec_funTW_volt_in/2(mot_ctrl_trs_trq_simu)
  parameter_selection/3(outport-mot_ctrl_cstr_trq_max_pos_simu-3) -> mot_ctrl_cmd_map_Pelec_funTW_volt_in/3(mot_ctrl_cstr_trq_max_pos_simu)
  parameter_selection/4(outport-mot_ctrl_cstr_trq_max_neg_simu-4) -> mot_ctrl_cmd_map_Pelec_funTW_volt_in/4(mot_ctrl_cstr_trq_max_neg_simu)
  aInport--2/1 -> Terminator_1/1
  aInport--3/1 -> Terminator_2/1
  aInport--4/1 -> Terminator_3/1

== system PowerSystemRefAeronomie/mot/ctrl/cstr ==
  inport-main_info_bus-1 : Inport
  aInport--2 : Inport  Port=2
  aInport--3 : Inport  Port=3
  Terminator_1 : Terminator
  Terminator_2 : Terminator
  mot_ctrl_cstr_map_Pelec_funTW_volt_in : Subsystem
  parameter_out : Subsystem
  parameter_selection : Subsystem
  outport-system_info_bus : Outport
  outport-cstr_bus : Outport  Port=2
  wires:
  inport-main_info_bus-1/1 -> parameter_selection/1(inport-main_info_bus-1)
  parameter_out/1(outport-system_info_bus) -> outport-system_info_bus/1
  parameter_out/2(outport-cstr_bus) -> outport-cstr_bus/1
  mot_ctrl_cstr_map_Pelec_funTW_volt_in/1(mot_ctrl_cstr_trq_pk_pos_simu) -> parameter_out/1(inport-mot_ctrl_cstr_trq_pk_pos_simu)
  mot_ctrl_cstr_map_Pelec_funTW_volt_in/2(mot_ctrl_cstr_trq_max_pos_simu) -> parameter_out/2(inport-mot_ctrl_cstr_trq_max_pos_simu)
  mot_ctrl_cstr_map_Pelec_funTW_volt_in/3(mot_ctrl_cstr_trq_pk_neg_simu) -> parameter_out/3(inport-mot_ctrl_cstr_trq_pk_neg_simu)
  mot_ctrl_cstr_map_Pelec_funTW_volt_in/4(mot_ctrl_cstr_trq_max_neg_simu) -> parameter_out/4(inport-mot_ctrl_cstr_trq_max_neg_simu)
  mot_ctrl_cstr_map_Pelec_funTW_volt_in/5(mot_ctrl_cstr_trq_cont_pos_simu) -> parameter_out/5(inport-mot_ctrl_cstr_trq_cont_pos_simu)
  mot_ctrl_cstr_map_Pelec_funTW_volt_in/6(mot_ctrl_cstr_trq_cont_neg_simu) -> parameter_out/6(inport-mot_ctrl_cstr_trq_cont_neg_simu)
  mot_ctrl_cstr_map_Pelec_funTW_volt_in/7(mot_ctrl_cstr_temp_coeff_simu) -> parameter_out/7(inport-mot_ctrl_cstr_temp_coeff_simu)
  parameter_selection/1(outport-mot_plant_spd_out_simu-1) -> mot_ctrl_cstr_map_Pelec_funTW_volt_in/1(mot_plant_spd_out_simu)
  parameter_selection/2(outport-mot_plant_temp_coeff_simu-2) -> mot_ctrl_cstr_map_Pelec_funTW_volt_in/2(mot_plant_temp_coeff_simu)
  aInport--2/1 -> Terminator_1/1
  aInport--3/1 -> Terminator_2/1

== system PowerSystemRefAeronomie/mot/ctrl/dmd ==
  inport-main_info_bus-1 : Inport
  aInport--2 : Inport  Port=2
  Terminator_1 : Terminator
  mot_ctrl_dmd_uas : Subsystem
  parameter_out : Subsystem
  parameter_selection : Subsystem
  outport-system_info_bus : Outport
  outport-dmd_bus : Outport  Port=2
  wires:
  parameter_selection/7(mot_plant_trq_out_simu) -> mot_ctrl_dmd_uas/7(mot_plant_trq_out_simu)
  parameter_selection/6(Vtas) -> mot_ctrl_dmd_uas/6(Vtas)
  inport-main_info_bus-1/1 -> parameter_selection/1(inport-main_info_bus-1)
  parameter_out/1(outport-system_info_bus) -> outport-system_info_bus/1
  parameter_out/2(outport-dmd_bus) -> outport-dmd_bus/1
  mot_ctrl_dmd_uas/1(mot_ctrl_trs_trq_simu) -> parameter_out/1(inport-mot_ctrl_trs_trq_simu)
  mot_ctrl_dmd_uas/2(mot_ctrl_ratedpwr_simu) -> parameter_out/2(inport-mot_ctrl_ratedpwr_simu)
  parameter_selection/1(outport-apc_ctrl_dt1_simu-1) -> mot_ctrl_dmd_uas/1(apc_ctrl_dt_simu)
  parameter_selection/2(outport-env_plant_density_simu-2) -> mot_ctrl_dmd_uas/2(env_plant_density_simu)
  parameter_selection/3(outport-ess_ctrl_pwr_max_pro_simu-3) -> mot_ctrl_dmd_uas/3(ess_ctrl_pwr_max_pro_simu)
  parameter_selection/4(outport-propel_plant_speed_simu-4) -> mot_ctrl_dmd_uas/4(propel_plant_speed_simu)
  parameter_selection/5(outport-tc_plant_spd_in_simu-5) -> mot_ctrl_dmd_uas/5(tc_plant_spd_in_simu)
  aInport--2/1 -> Terminator_1/1

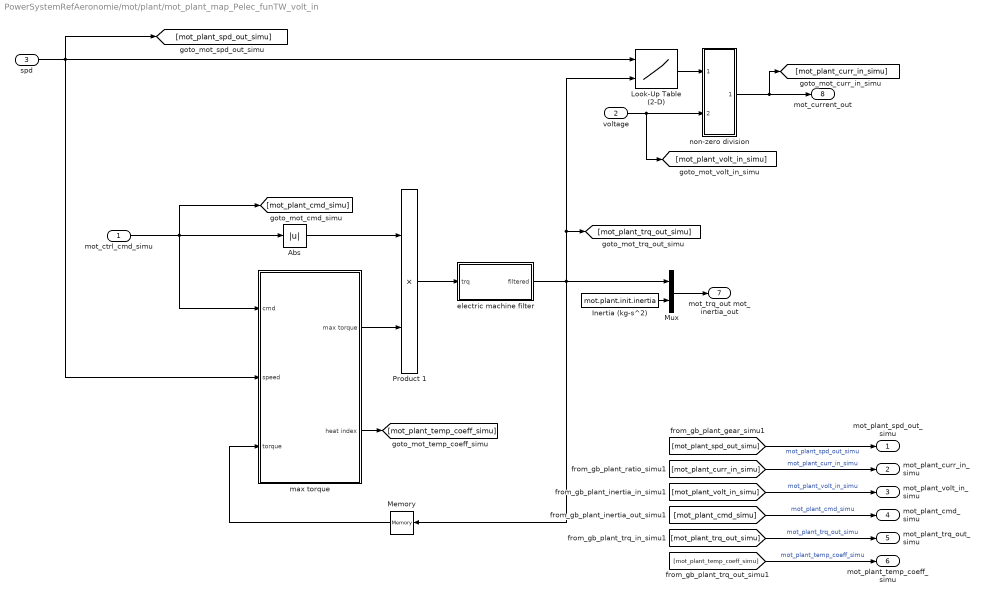
== system PowerSystemRefAeronomie/mot/plant/mot_plant_map_Pelec_funTW_volt_in ==
  mot_ctrl_cmd_simu : Inport
  voltage : Inport  Port=2
  spd : Inport  Port=3
  Abs : Abs
  Inertia (kg-s^2) : Constant  Value=mot.plant.init.inertia
  Look-Up Table (2-D) : Lookup2D  RowIndex=mot.plant.calc.pwr_elec.idx1_spd  ColumnIndex=mot.plant.calc.pwr_elec.idx2_trq  Table=mot.plant.calc.pwr_elec.map
  Memory : Memory
  Mux : Mux  Inputs=2
  Product 1 : Product  InputSameDT=on  SaturateOnIntegerOverflow=on  OutDataTypeStr=Inherit: Same as first input
  electric machine filter : Subsystem
  "max torque " : Subsystem
  non-zero division : Subsystem
      mask Display: disp('divider \n I1/I2')
  mot_plant_spd_out_simu : Outport
  mot_plant_curr_in_simu : Outport  Port=2
  mot_plant_volt_in_simu : Outport  Port=3
  mot_plant_cmd_simu : Outport  Port=4
  mot_plant_trq_out_simu : Outport  Port=5
  mot_plant_temp_coeff_simu : Outport  Port=6
  mot_trq_out mot_inertia_out : Outport  Port=7
  mot_current_out : Outport  Port=8
  wires:
  Look-Up Table (2-D)/1 -> non-zero division/1(In1)
  [mot_plant_temp_coeff_simu] -> mot_plant_temp_coeff_simu/1  "mot_plant_temp_coeff_simu"
  [mot_plant_trq_out_simu] -> mot_plant_trq_out_simu/1  "mot_plant_trq_out_simu"
  [mot_plant_cmd_simu] -> mot_plant_cmd_simu/1  "mot_plant_cmd_simu"
  [mot_plant_volt_in_simu] -> mot_plant_volt_in_simu/1  "mot_plant_volt_in_simu"
  [mot_plant_curr_in_simu] -> mot_plant_curr_in_simu/1  "mot_plant_curr_in_simu"
  [mot_plant_spd_out_simu] -> mot_plant_spd_out_simu/1  "mot_plant_spd_out_simu"
  electric machine filter/1(filtered) -> Mux/1, Memory/1, [mot_plant_trq_out_simu], Look-Up Table (2-D)/2
  "max torque "/1(max torque) -> Product 1/2
  Product 1/1 -> electric machine filter/1(trq)
  Abs/1 -> Product 1/1
  Memory/1 -> "max torque "/3(torque)
  mot_ctrl_cmd_simu/1 -> "max torque "/1(cmd), [mot_plant_cmd_simu], Abs/1
  Inertia (kg-s^2)/1 -> Mux/2
  Mux/1 -> mot_trq_out mot_inertia_out/1
  spd/1 -> [mot_plant_spd_out_simu], "max torque "/2(speed), Look-Up Table (2-D)/1
  "max torque "/2(heat index) -> [mot_plant_temp_coeff_simu]
  non-zero division/1(Out1) -> mot_current_out/1, [mot_plant_curr_in_simu]
  voltage/1 -> non-zero division/2(In2), [mot_plant_volt_in_simu]

== system PowerSystemRefAeronomie/mot/plant/parameter_out ==
  inport-mot_plant_spd_out_simu : Inport
  inport-mot_plant_curr_in_simu : Inport  Port=2
  inport-mot_plant_volt_in_simu : Inport  Port=3
  inport-mot_plant_cmd_simu : Inport  Port=4
  inport-mot_plant_trq_out_simu : Inport  Port=5
  inport-mot_plant_temp_coeff_simu : Inport  Port=6
  Ground_1 : Ground
  Toworkspace-mot_plant_cmd_simu : ToWorkspace  VariableName=mot_plant_cmd_simu  SampleTime=pxf_diagram_options.workspace_sample_time
      settings: Decimation=pxf_diagram_options.decimation
  Toworkspace-mot_plant_curr_in_simu : ToWorkspace  VariableName=mot_plant_curr_in_simu  SampleTime=pxf_diagram_options.workspace_sample_time
      settings: Decimation=pxf_diagram_options.decimation
  Toworkspace-mot_plant_spd_out_simu : ToWorkspace  VariableName=mot_plant_spd_out_simu  SampleTime=pxf_diagram_options.workspace_sample_time
      settings: Decimation=pxf_diagram_options.decimation
  Toworkspace-mot_plant_temp_coeff_simu : ToWorkspace  VariableName=mot_plant_temp_coeff_simu  SampleTime=pxf_diagram_options.workspace_sample_time
      settings: Decimation=pxf_diagram_options.decimation
  Toworkspace-mot_plant_trq_out_simu : ToWorkspace  VariableName=mot_plant_trq_out_simu  SampleTime=pxf_diagram_options.workspace_sample_time
      settings: Decimation=pxf_diagram_options.decimation
  Toworkspace-mot_plant_volt_in_simu : ToWorkspace  VariableName=mot_plant_volt_in_simu  SampleTime=pxf_diagram_options.workspace_sample_time
      settings: Decimation=pxf_diagram_options.decimation
  create_system_info_bus : BusCreator  Inputs=3
  outport-system_info_bus : Outport
  outport-plant_bus : Outport  Port=2
  wires:
  create_system_info_bus/1 -> outport-system_info_bus/1
  inport-mot_plant_spd_out_simu/1 -> create_system_info_bus/1, Toworkspace-mot_plant_spd_out_simu/1  "mot_plant_spd_out_simu"
  inport-mot_plant_curr_in_simu/1 -> Toworkspace-mot_plant_curr_in_simu/1
  inport-mot_plant_volt_in_simu/1 -> Toworkspace-mot_plant_volt_in_simu/1
  inport-mot_plant_cmd_simu/1 -> Toworkspace-mot_plant_cmd_simu/1
  inport-mot_plant_trq_out_simu/1 -> create_system_info_bus/3, Toworkspace-mot_plant_trq_out_simu/1
  inport-mot_plant_temp_coeff_simu/1 -> create_system_info_bus/2, Toworkspace-mot_plant_temp_coeff_simu/1  "mot_plant_temp_coeff_simu"
  Ground_1/1 -> outport-plant_bus/1

== system PowerSystemRefAeronomie/mot/plant/parameter_selection ==
  Inport_1 : Inport
  inport-ctrl_bus-2 : Inport  Port=2
  Terminator_1 : Terminator
  select_ctrl_bus : BusSelector  OutputSignals=mot_ctrl_cmd_simu
  outport-mot_ctrl_cmd_simu-1 : Outport
  wires:
  inport-ctrl_bus-2/1 -> select_ctrl_bus/1
  select_ctrl_bus/1 -> outport-mot_ctrl_cmd_simu-1/1  "<mot_ctrl_cmd_simu>"
  Inport_1/1 -> Terminator_1/1

== system PowerSystemRefAeronomie/propel/plant/parameter_out ==
  inport-propel_plant_speed_simu : Inport
  inport-propel_plant_pwr_in_simu : Inport  Port=2
  inport-propel_plant_pwr_out_simu : Inport  Port=3
  inport-propel_plant_thrust_simu : Inport  Port=4
  propel_plant_effort : Inport  Port=5
  propel_plant_effort_dn1 : Inport  Port=6
  Toworkspace-propel_plant_pwr_in_simu : ToWorkspace  VariableName=propel_plant_pwr_in_simu  SampleTime=pxf_diagram_options.workspace_sample_time
      settings: Decimation=pxf_diagram_options.decimation
  Toworkspace-propel_plant_pwr_out_simu : ToWorkspace  VariableName=propel_plant_pwr_out_simu  SampleTime=pxf_diagram_options.workspace_sample_time
      settings: Decimation=pxf_diagram_options.decimation
  Toworkspace-propel_plant_speed_simu : ToWorkspace  VariableName=propel_plant_speed_simu  SampleTime=pxf_diagram_options.workspace_sample_time
      settings: Decimation=pxf_diagram_options.decimation
  Toworkspace-propel_plant_thrust_simu : ToWorkspace  VariableName=propel_plant_thrust_simu  SampleTime=pxf_diagram_options.workspace_sample_time
      settings: Decimation=pxf_diagram_options.decimation
  create_system_info_bus : BusCreator  Commented=on  Inputs=1
  create_system_info_bus1 : BusCreator  Inputs=3
  outport-system_info_bus : Outport
  wires:
  create_system_info_bus1/1 -> outport-system_info_bus/1
  propel_plant_effort/1 -> create_system_info_bus1/2
  propel_plant_effort_dn1/1 -> create_system_info_bus1/3  "propel_plant_effort_dn"
  inport-propel_plant_speed_simu/1 -> create_system_info_bus/1, Toworkspace-propel_plant_speed_simu/1, create_system_info_bus1/1  "propel_plant_speed_simu"
  inport-propel_plant_pwr_in_simu/1 -> Toworkspace-propel_plant_pwr_in_simu/1
  inport-propel_plant_pwr_out_simu/1 -> Toworkspace-propel_plant_pwr_out_simu/1
  inport-propel_plant_thrust_simu/1 -> Toworkspace-propel_plant_thrust_simu/1
